simulink model "monocopter_sim"  (R2026a)
settings: Solver=ode4  StopTime=10  FixedStep=Ts
undefined symbols (not defined in the file): alt_ref_const, b_aero, b_pitch, b_roll, c_q, F_to_throttle, g, Ixx, Iyy, Izz, joy_pitch_const, joy_roll_const, kappa_y, Kd_alt, Kd_pitch, Kd_roll, Kd_yaw, Ki_alt, Ki_pitch, Ki_roll, Ki_yaw, Kp_alt, Kp_pitch, Kp_roll, Kp_yaw, Ks_hover, kT, Ky_hover, m, mode_const, omega_hover, omega_max, pid_alt_force_max, pid_alt_int_max, pid_pitch_int_max, pid_pitch_torque_max, pid_roll_int_max, pid_roll_torque_max, pid_yaw_int_max, pid_yaw_torque_max, servo_max, servo_min, throttle_const, Ts, yaw_ff, yaw_ref_const
libraries: slpidlib x4, simulink x4
settings Model: Creator=macbookpro
settings DataIOCC: SaveState=on

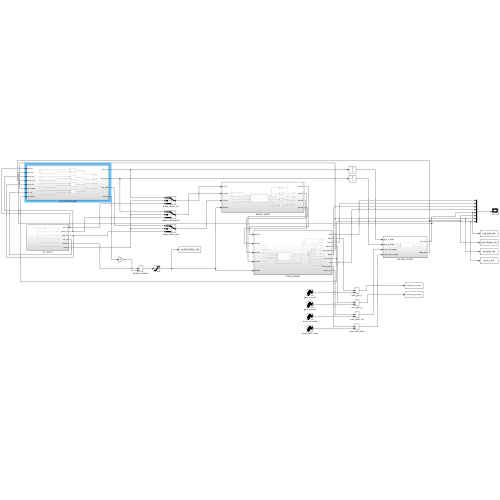
[thumbnail: Simulink's stored preview of the top-level diagram]
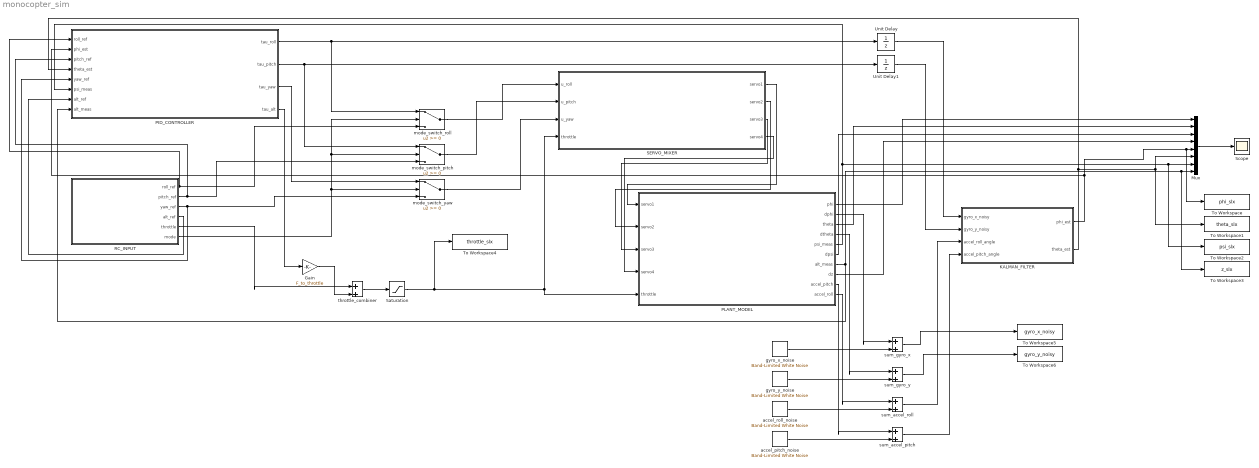
== system monocopter_sim ==
  Gain : Gain  Gain=F_to_throttle
  KALMAN_FILTER : Subsystem
  Mux : Mux  Inputs=8
  PID_CONTROLLER : Subsystem
  PLANT_MODEL : Subsystem
  RC_INPUT : Subsystem
  SERVO_MIXER : Subsystem
  Saturation : Saturate  UpperLimit=1  LowerLimit=0.05
  Scope : Scope
      settings: ActiveDisplayYMinimum=-8.14946670637509E+7  ActiveDisplayYMaximum=9.2907040776445866E+7
  To Workspace : ToWorkspace  VariableName=phi_slx  SaveFormat=Timeseries  SampleTime=-1
  To Workspace1 : ToWorkspace  VariableName=theta_slx  SaveFormat=Timeseries  SampleTime=-1
  To Workspace2 : ToWorkspace  VariableName=psi_slx  SaveFormat=Timeseries  SampleTime=-1
  To Workspace3 : ToWorkspace  VariableName=z_slx  SaveFormat=Timeseries  SampleTime=-1
  To Workspace4 : ToWorkspace  VariableName=throttle_slx  SaveFormat=Timeseries  SampleTime=-1
  To Workspace5 : ToWorkspace  VariableName=gyro_x_noisy  SaveFormat=Timeseries  SampleTime=-1
  To Workspace6 : ToWorkspace  VariableName=gyro_y_noisy  SaveFormat=Timeseries  SampleTime=-1
  Unit Delay : UnitDelay  SampleTime=Ts
  Unit Delay1 : UnitDelay  SampleTime=Ts
  "accel_pitch_noise " : simulink/Sources/Band-Limited White Noise  Cov=accel_noise_sim  Ts=Ts  seed=noise_seed_ap
  accel_roll_noise : simulink/Sources/Band-Limited White Noise  Cov=accel_noise_sim  Ts=Ts  seed=noise_seed_ar
  gyro_x_noise : simulink/Sources/Band-Limited White Noise  Cov=gyro_noise_sim  Ts=Ts  seed=noise_seed_gx
  gyro_y_noise : simulink/Sources/Band-Limited White Noise  Cov=gyro_noise_sim  Ts=Ts  seed=noise_seed_gy
  mode_switch_pitch : Switch  SaturateOnIntegerOverflow=off  InputSameDT=off
  mode_switch_roll : Switch  SaturateOnIntegerOverflow=off  InputSameDT=off
  mode_switch_yaw : Switch  SaturateOnIntegerOverflow=off  InputSameDT=off
  sum_accel_pitch : Sum  Inputs=|++
  sum_accel_roll : Sum  Inputs=|++
  sum_gyro_x : Sum  Inputs=|++
  sum_gyro_y : Sum  Inputs=|++
  throttle_combiner : Sum  Inputs=|++
  wires:
  PLANT_MODEL/2(dphi) -> sum_gyro_x/1
  gyro_x_noise/1 -> sum_gyro_x/2
  PLANT_MODEL/4(dtheta) -> sum_gyro_y/1
  gyro_y_noise/1 -> sum_gyro_y/2
  PLANT_MODEL/10(accel_roll) -> sum_accel_roll/1
  accel_roll_noise/1 -> sum_accel_roll/2
  PLANT_MODEL/9(accel_pitch) -> sum_accel_pitch/1
  "accel_pitch_noise "/1 -> sum_accel_pitch/2
  sum_accel_roll/1 -> KALMAN_FILTER/3(accel_roll_angle)
  sum_accel_pitch/1 -> KALMAN_FILTER/4(accel_pitch_angle)
  PID_CONTROLLER/1(tau_roll) -> Unit Delay/1, mode_switch_roll/1
  RC_INPUT/6(mode) -> mode_switch_yaw/2, mode_switch_roll/2, mode_switch_pitch/2
  RC_INPUT/1(roll_ref) -> PID_CONTROLLER/1(roll_ref), mode_switch_roll/3
  mode_switch_roll/1 -> SERVO_MIXER/1(u_roll)
  mode_switch_pitch/1 -> SERVO_MIXER/2(u_pitch)
  mode_switch_yaw/1 -> SERVO_MIXER/3(u_yaw)
  PID_CONTROLLER/2(tau_pitch) -> Unit Delay1/1, mode_switch_pitch/1
  PID_CONTROLLER/3(tau_yaw) -> mode_switch_yaw/1
  RC_INPUT/2(pitch_ref) -> PID_CONTROLLER/3(pitch_ref), mode_switch_pitch/3
  RC_INPUT/3(yaw_ref) -> PID_CONTROLLER/5(yaw_ref), mode_switch_yaw/3
  RC_INPUT/5(throttle) -> throttle_combiner/1
  RC_INPUT/4(alt_ref) -> PID_CONTROLLER/7(alt_ref)
  KALMAN_FILTER/1(phi_est) -> PID_CONTROLLER/2(phi_est), To Workspace/1, Mux/5
  KALMAN_FILTER/2(theta_est) -> Mux/6, To Workspace1/1, PID_CONTROLLER/4(theta_est)
  SERVO_MIXER/1(servo1) -> PLANT_MODEL/1(servo1)
  SERVO_MIXER/2(servo2) -> PLANT_MODEL/2(servo2)
  SERVO_MIXER/3(servo3) -> PLANT_MODEL/3(servo3)
  SERVO_MIXER/4(servo4) -> PLANT_MODEL/4(servo4)
  PLANT_MODEL/5(psi_meas) -> Mux/7, To Workspace2/1, PID_CONTROLLER/6(psi_meas)
  PLANT_MODEL/7(alt_meas) -> Mux/8, To Workspace3/1, PID_CONTROLLER/8(alt_meas)
  PLANT_MODEL/3(theta) -> Mux/2
  PLANT_MODEL/6(dpsi) -> Mux/3
  PLANT_MODEL/8(dz) -> Mux/4
  Mux/1 -> Scope/1
  PLANT_MODEL/1(phi) -> Mux/1
  throttle_combiner/1 -> Saturation/1
  Saturation/1 -> PLANT_MODEL/5(throttle), SERVO_MIXER/4(throttle), To Workspace4/1
  sum_gyro_y/1 -> To Workspace6/1
  PID_CONTROLLER/4(tau_alt) -> Gain/1
  Gain/1 -> throttle_combiner/2
  Unit Delay1/1 -> KALMAN_FILTER/2(gyro_y_noisy)
  sum_gyro_x/1 -> To Workspace5/1
  Unit Delay/1 -> KALMAN_FILTER/1(gyro_x_noisy)

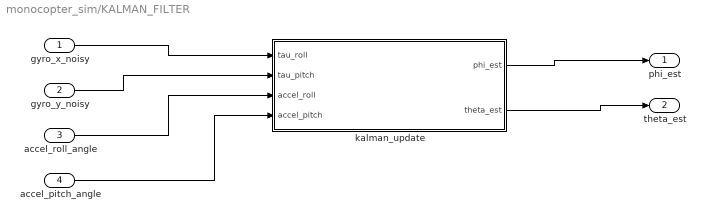
== system monocopter_sim/KALMAN_FILTER ==
  gyro_x_noisy : Inport
  gyro_y_noisy : Inport  Port=2
  accel_roll_angle : Inport  Port=3
  accel_pitch_angle : Inport  Port=4
  kalman_update : MATLAB Function  TreatAsAtomicUnit=on  SystemSampleTime=Ts
  phi_est : Outport
  theta_est : Outport  Port=2
  wires:
  gyro_x_noisy/1 -> kalman_update/1(tau_roll)
  gyro_y_noisy/1 -> kalman_update/2(tau_pitch)
  accel_roll_angle/1 -> kalman_update/3(accel_roll)
  accel_pitch_angle/1 -> kalman_update/4(accel_pitch)
  kalman_update/1(phi_est) -> phi_est/1
  kalman_update/2(theta_est) -> theta_est/1

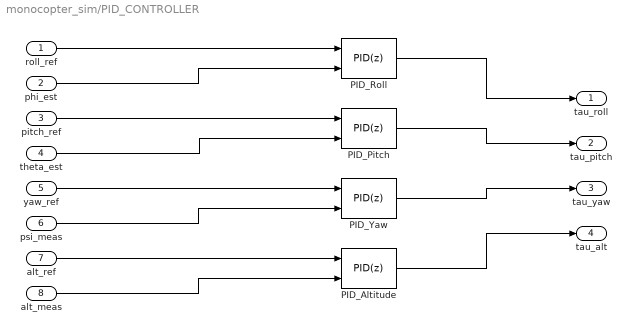
== system monocopter_sim/PID_CONTROLLER ==
  roll_ref : Inport
  phi_est : Inport  Port=2
  pitch_ref : Inport  Port=3
  theta_est : Inport  Port=4
  yaw_ref : Inport  Port=5
  psi_meas : Inport  Port=6
  alt_ref : Inport  Port=7
  alt_meas : Inport  Port=8
  PID_Altitude : slpidlib/PID Controller (2DOF)  Controller=PID  Form=Parallel  TimeDomain=Discrete-time  UseExternalTs=off  SampleTime=Ts  IntegratorMethod=Forward Euler  FilterMethod=Forward Euler  ControllerParametersSource=internal  P=Kp_alt  I=Ki_alt  UseKiTs=off  D=Kd_alt  UseExternalDerivativeSource=off  N=100  UseFilter=on  b=0  c=0  TunerSelectOption=Transfer Function Based (PID Tuner App)  InitialConditionSource=internal  InitialConditionForIntegrator=0  InitialConditionForFilter=0  DifferentiatorICPrevScaledInput=0  ExternalReset=none  TrackingMode=off  Kt=1  LimitOutput=on  SatLimitsSource=internal  UpperSaturationLimit=pid_alt_force_max  LowerSaturationLimit=-pid_alt_force_max  LinearizeAsGain=on  AntiWindupMode=clamping  Kb=1  LimitIntegrator=on  UpperIntegratorSaturationLimit=pid_alt_int_max  LowerIntegratorSaturationLimit=-pid_alt_int_max  POutMin=[]  POutMax=[]  IOutMin=[]  IOutMax=[]  DOutMin=[]  DOutMax=[]  NOutMin=[]  NOutMax=[]  bOutMin=[]  bOutMax=[]  cOutMin=[]  cOutMax=[]  SumOutMin=[]  SumOutMax=[]  SaturationOutMin=[]  SaturationOutMax=[]  PParamMin=[]  PParamMax=[]  IParamMin=[]  IParamMax=[]  DParamMin=[]  DParamMax=[]  NParamMin=[]  NParamMax=[]  bParamMin=[]  bParamMax=[]  cParamMin=[]  cParamMax=[]  KbParamMin=[]  KbParamMax=[]  KtParamMin=[]  KtParamMax=[]  KbOutMin=[]  KbOutMax=[]  KtOutMin=[]  KtOutMax=[]  IntegratorOutMin=[]  IntegratorOutMax=[]  FilterOutMin=[]  FilterOutMax=[]  SumI1OutMin=[]  SumI1OutMax=[]  SumI2OutMin=[]  SumI2OutMax=[]  SumI3OutMin=[]  SumI3OutMax=[]  SumI4OutMin=[]  SumI4OutMax=[]  SumDOutMin=[]  SumDOutMax=[]  Sum1OutMin=[]  Sum1OutMax=[]  Sum2OutMin=[]  Sum2OutMax=[]  Sum3OutMin=[]  Sum3OutMax=[]  DifferentiatorOutMin=[]  DifferentiatorOutMax=[]  FilterDiffOutCoefMin=[]  FilterDiffOutCoefMax=[]  ReciprocalOutMin=[]  ReciprocalOutMax=[]  SumDenOutMin=[]  SumDenOutMax=[]  SumNumOutMin=[]  SumNumOutMax=[]  DivideOutMin=[]  DivideOutMax=[]  UdiffTsProdOutMin=[]  UdiffTsProdOutMax=[]  NTsProdOutMin=[]  NTsProdOutMax=[]  UintegralTsProdOutMin=[]  UintegralTsProdOutMax=[]  UngainTsProdOutMin=[]  UngainTsProdOutMax=[]  ClampingZeroOutDataTypeStr=Inherit: Inherit via back propagation  ClampingZeroOutMin=[]  ClampingZeroOutMax=[]  FilterDenConstantOutDataTypeStr=Inherit: Inherit via back propagation  FilterDenConstantOutMin=[]  FilterDenConstantOutMax=[]  PCopyOutDataTypeStr=Inherit: Inherit via back propagation  PCopyOutMin=[]  PCopyOutMax=[]  NCopyOutDataTypeStr=Inherit: Inherit via back propagation  NCopyOutMin=[]  NCopyOutMax=[]  IntegratorContinuousStateAttributes=''  IntegratorStateMustResolveToSignalObject=off  IntegratorRTWStateStorageClass=Auto  FilterContinuousStateAttributes=''  FilterStateMustResolveToSignalObject=off  FilterRTWStateStorageClass=Auto  ParallelPVariant=InternalParameters  IdealPVariant=Disabled  IVariant=InternalParameters  DVariant=InternalParameters  bVariant=InternalParameters  cVariant=InternalParameters  IntegratorVariant=Discrete  SatVariant=Enabled  AWVariant=DiscClampingParallel  PCopyVariant=Disabled  TRVariant=Disabled  FdbkBlocksVariant=Forward  IdealPFdbkVariant=Disabled  SatFdbkVariant=Disabled  DerivativeFilterVariant=ForwardEulerFilter  NVariant=InternalParameters  NCopyVariant=Disabled  FilterICVariant=InternalICsFilter  IntegratorICVariant=InternalICs  ExternalResetVariant=Disabled  TRSumVariant=Passthrough  SumFdbkVariant=Disabled  SumVariant=Sum_PID  TsampFilterVariant=InternalTs  TsampNgainVariant=Passthrough  TsampIntegralVariant=Disabled_SignalSpec  ExternalSaturationOutDataTypeStr=Inherit: Same as second input  DerivativeSourceVariant=ErrorSignal  PreIntVariant=InternalPreInt
  PID_Pitch : slpidlib/PID Controller (2DOF)  Controller=PID  Form=Parallel  TimeDomain=Discrete-time  UseExternalTs=off  SampleTime=Ts  IntegratorMethod=Forward Euler  FilterMethod=Forward Euler  ControllerParametersSource=internal  P=Kp_pitch  I=Ki_pitch  UseKiTs=off  D=Kd_pitch  UseExternalDerivativeSource=off  N=100  UseFilter=on  b=0  c=0  TunerSelectOption=Transfer Function Based (PID Tuner App)  InitialConditionSource=internal  InitialConditionForIntegrator=0  InitialConditionForFilter=0  DifferentiatorICPrevScaledInput=0  ExternalReset=none  TrackingMode=off  Kt=1  LimitOutput=on  SatLimitsSource=internal  UpperSaturationLimit=pid_pitch_torque_max  LowerSaturationLimit=-pid_pitch_torque_max  LinearizeAsGain=on  AntiWindupMode=clamping  Kb=1  LimitIntegrator=on  UpperIntegratorSaturationLimit=pid_pitch_int_max  LowerIntegratorSaturationLimit=-pid_pitch_int_max  POutMin=[]  POutMax=[]  IOutMin=[]  IOutMax=[]  DOutMin=[]  DOutMax=[]  NOutMin=[]  NOutMax=[]  bOutMin=[]  bOutMax=[]  cOutMin=[]  cOutMax=[]  SumOutMin=[]  SumOutMax=[]  SaturationOutMin=[]  SaturationOutMax=[]  PParamMin=[]  PParamMax=[]  IParamMin=[]  IParamMax=[]  DParamMin=[]  DParamMax=[]  NParamMin=[]  NParamMax=[]  bParamMin=[]  bParamMax=[]  cParamMin=[]  cParamMax=[]  KbParamMin=[]  KbParamMax=[]  KtParamMin=[]  KtParamMax=[]  KbOutMin=[]  KbOutMax=[]  KtOutMin=[]  KtOutMax=[]  IntegratorOutMin=[]  IntegratorOutMax=[]  FilterOutMin=[]  FilterOutMax=[]  SumI1OutMin=[]  SumI1OutMax=[]  SumI2OutMin=[]  SumI2OutMax=[]  SumI3OutMin=[]  SumI3OutMax=[]  SumI4OutMin=[]  SumI4OutMax=[]  SumDOutMin=[]  SumDOutMax=[]  Sum1OutMin=[]  Sum1OutMax=[]  Sum2OutMin=[]  Sum2OutMax=[]  Sum3OutMin=[]  Sum3OutMax=[]  DifferentiatorOutMin=[]  DifferentiatorOutMax=[]  FilterDiffOutCoefMin=[]  FilterDiffOutCoefMax=[]  ReciprocalOutMin=[]  ReciprocalOutMax=[]  SumDenOutMin=[]  SumDenOutMax=[]  SumNumOutMin=[]  SumNumOutMax=[]  DivideOutMin=[]  DivideOutMax=[]  UdiffTsProdOutMin=[]  UdiffTsProdOutMax=[]  NTsProdOutMin=[]  NTsProdOutMax=[]  UintegralTsProdOutMin=[]  UintegralTsProdOutMax=[]  UngainTsProdOutMin=[]  UngainTsProdOutMax=[]  ClampingZeroOutDataTypeStr=Inherit: Inherit via back propagation  ClampingZeroOutMin=[]  ClampingZeroOutMax=[]  FilterDenConstantOutDataTypeStr=Inherit: Inherit via back propagation  FilterDenConstantOutMin=[]  FilterDenConstantOutMax=[]  PCopyOutDataTypeStr=Inherit: Inherit via back propagation  PCopyOutMin=[]  PCopyOutMax=[]  NCopyOutDataTypeStr=Inherit: Inherit via back propagation  NCopyOutMin=[]  NCopyOutMax=[]  IntegratorContinuousStateAttributes=''  IntegratorStateMustResolveToSignalObject=off  IntegratorRTWStateStorageClass=Auto  FilterContinuousStateAttributes=''  FilterStateMustResolveToSignalObject=off  FilterRTWStateStorageClass=Auto  ParallelPVariant=InternalParameters  IdealPVariant=Disabled  IVariant=InternalParameters  DVariant=InternalParameters  bVariant=InternalParameters  cVariant=InternalParameters  IntegratorVariant=Discrete  SatVariant=Enabled  AWVariant=DiscClampingParallel  PCopyVariant=Disabled  TRVariant=Disabled  FdbkBlocksVariant=Forward  IdealPFdbkVariant=Disabled  SatFdbkVariant=Disabled  DerivativeFilterVariant=ForwardEulerFilter  NVariant=InternalParameters  NCopyVariant=Disabled  FilterICVariant=InternalICsFilter  IntegratorICVariant=InternalICs  ExternalResetVariant=Disabled  TRSumVariant=Passthrough  SumFdbkVariant=Disabled  SumVariant=Sum_PID  TsampFilterVariant=InternalTs  TsampNgainVariant=Passthrough  TsampIntegralVariant=Disabled_SignalSpec  ExternalSaturationOutDataTypeStr=Inherit: Same as second input  DerivativeSourceVariant=ErrorSignal  PreIntVariant=InternalPreInt
  PID_Roll : slpidlib/PID Controller (2DOF)  Controller=PID  Form=Parallel  TimeDomain=Discrete-time  UseExternalTs=off  SampleTime=Ts  IntegratorMethod=Forward Euler  FilterMethod=Forward Euler  ControllerParametersSource=internal  P=Kp_roll  I=Ki_roll  UseKiTs=off  D=Kd_roll  UseExternalDerivativeSource=off  N=100  UseFilter=on  b=0  c=0  TunerSelectOption=Transfer Function Based (PID Tuner App)  InitialConditionSource=internal  InitialConditionForIntegrator=0  InitialConditionForFilter=0  DifferentiatorICPrevScaledInput=0  ExternalReset=none  TrackingMode=off  Kt=1  LimitOutput=on  SatLimitsSource=internal  UpperSaturationLimit=pid_roll_torque_max  LowerSaturationLimit=-pid_roll_torque_max  LinearizeAsGain=on  AntiWindupMode=clamping  Kb=1  LimitIntegrator=on  UpperIntegratorSaturationLimit=pid_roll_int_max  LowerIntegratorSaturationLimit=-pid_roll_int_max  POutMin=[]  POutMax=[]  IOutMin=[]  IOutMax=[]  DOutMin=[]  DOutMax=[]  NOutMin=[]  NOutMax=[]  bOutMin=[]  bOutMax=[]  cOutMin=[]  cOutMax=[]  SumOutMin=[]  SumOutMax=[]  SaturationOutMin=[]  SaturationOutMax=[]  PParamMin=[]  PParamMax=[]  IParamMin=[]  IParamMax=[]  DParamMin=[]  DParamMax=[]  NParamMin=[]  NParamMax=[]  bParamMin=[]  bParamMax=[]  cParamMin=[]  cParamMax=[]  KbParamMin=[]  KbParamMax=[]  KtParamMin=[]  KtParamMax=[]  KbOutMin=[]  KbOutMax=[]  KtOutMin=[]  KtOutMax=[]  IntegratorOutMin=[]  IntegratorOutMax=[]  FilterOutMin=[]  FilterOutMax=[]  SumI1OutMin=[]  SumI1OutMax=[]  SumI2OutMin=[]  SumI2OutMax=[]  SumI3OutMin=[]  SumI3OutMax=[]  SumI4OutMin=[]  SumI4OutMax=[]  SumDOutMin=[]  SumDOutMax=[]  Sum1OutMin=[]  Sum1OutMax=[]  Sum2OutMin=[]  Sum2OutMax=[]  Sum3OutMin=[]  Sum3OutMax=[]  DifferentiatorOutMin=[]  DifferentiatorOutMax=[]  FilterDiffOutCoefMin=[]  FilterDiffOutCoefMax=[]  ReciprocalOutMin=[]  ReciprocalOutMax=[]  SumDenOutMin=[]  SumDenOutMax=[]  SumNumOutMin=[]  SumNumOutMax=[]  DivideOutMin=[]  DivideOutMax=[]  UdiffTsProdOutMin=[]  UdiffTsProdOutMax=[]  NTsProdOutMin=[]  NTsProdOutMax=[]  UintegralTsProdOutMin=[]  UintegralTsProdOutMax=[]  UngainTsProdOutMin=[]  UngainTsProdOutMax=[]  ClampingZeroOutDataTypeStr=Inherit: Inherit via back propagation  ClampingZeroOutMin=[]  ClampingZeroOutMax=[]  FilterDenConstantOutDataTypeStr=Inherit: Inherit via back propagation  FilterDenConstantOutMin=[]  FilterDenConstantOutMax=[]  PCopyOutDataTypeStr=Inherit: Inherit via back propagation  PCopyOutMin=[]  PCopyOutMax=[]  NCopyOutDataTypeStr=Inherit: Inherit via back propagation  NCopyOutMin=[]  NCopyOutMax=[]  IntegratorContinuousStateAttributes=''  IntegratorStateMustResolveToSignalObject=off  IntegratorRTWStateStorageClass=Auto  FilterContinuousStateAttributes=''  FilterStateMustResolveToSignalObject=off  FilterRTWStateStorageClass=Auto  ParallelPVariant=InternalParameters  IdealPVariant=Disabled  IVariant=InternalParameters  DVariant=InternalParameters  bVariant=InternalParameters  cVariant=InternalParameters  IntegratorVariant=Discrete  SatVariant=Enabled  AWVariant=DiscClampingParallel  PCopyVariant=Disabled  TRVariant=Disabled  FdbkBlocksVariant=Forward  IdealPFdbkVariant=Disabled  SatFdbkVariant=Disabled  DerivativeFilterVariant=ForwardEulerFilter  NVariant=InternalParameters  NCopyVariant=Disabled  FilterICVariant=InternalICsFilter  IntegratorICVariant=InternalICs  ExternalResetVariant=Disabled  TRSumVariant=Passthrough  SumFdbkVariant=Disabled  SumVariant=Sum_PID  TsampFilterVariant=InternalTs  TsampNgainVariant=Passthrough  TsampIntegralVariant=Disabled_SignalSpec  ExternalSaturationOutDataTypeStr=Inherit: Same as second input  DerivativeSourceVariant=ErrorSignal  PreIntVariant=InternalPreInt
  PID_Yaw : slpidlib/PID Controller (2DOF)  Controller=PID  Form=Parallel  TimeDomain=Discrete-time  UseExternalTs=off  SampleTime=Ts  IntegratorMethod=Forward Euler  FilterMethod=Forward Euler  ControllerParametersSource=internal  P=Kp_yaw  I=Ki_yaw  UseKiTs=off  D=Kd_yaw  UseExternalDerivativeSource=off  N=100  UseFilter=on  b=0  c=0  TunerSelectOption=Transfer Function Based (PID Tuner App)  InitialConditionSource=internal  InitialConditionForIntegrator=0  InitialConditionForFilter=0  DifferentiatorICPrevScaledInput=0  ExternalReset=none  TrackingMode=off  Kt=1  LimitOutput=on  SatLimitsSource=internal  UpperSaturationLimit=pid_yaw_torque_max  LowerSaturationLimit=-pid_yaw_torque_max  LinearizeAsGain=on  AntiWindupMode=clamping  Kb=1  LimitIntegrator=on  UpperIntegratorSaturationLimit=pid_yaw_int_max  LowerIntegratorSaturationLimit=-pid_yaw_int_max  POutMin=[]  POutMax=[]  IOutMin=[]  IOutMax=[]  DOutMin=[]  DOutMax=[]  NOutMin=[]  NOutMax=[]  bOutMin=[]  bOutMax=[]  cOutMin=[]  cOutMax=[]  SumOutMin=[]  SumOutMax=[]  SaturationOutMin=[]  SaturationOutMax=[]  PParamMin=[]  PParamMax=[]  IParamMin=[]  IParamMax=[]  DParamMin=[]  DParamMax=[]  NParamMin=[]  NParamMax=[]  bParamMin=[]  bParamMax=[]  cParamMin=[]  cParamMax=[]  KbParamMin=[]  KbParamMax=[]  KtParamMin=[]  KtParamMax=[]  KbOutMin=[]  KbOutMax=[]  KtOutMin=[]  KtOutMax=[]  IntegratorOutMin=[]  IntegratorOutMax=[]  FilterOutMin=[]  FilterOutMax=[]  SumI1OutMin=[]  SumI1OutMax=[]  SumI2OutMin=[]  SumI2OutMax=[]  SumI3OutMin=[]  SumI3OutMax=[]  SumI4OutMin=[]  SumI4OutMax=[]  SumDOutMin=[]  SumDOutMax=[]  Sum1OutMin=[]  Sum1OutMax=[]  Sum2OutMin=[]  Sum2OutMax=[]  Sum3OutMin=[]  Sum3OutMax=[]  DifferentiatorOutMin=[]  DifferentiatorOutMax=[]  FilterDiffOutCoefMin=[]  FilterDiffOutCoefMax=[]  ReciprocalOutMin=[]  ReciprocalOutMax=[]  SumDenOutMin=[]  SumDenOutMax=[]  SumNumOutMin=[]  SumNumOutMax=[]  DivideOutMin=[]  DivideOutMax=[]  UdiffTsProdOutMin=[]  UdiffTsProdOutMax=[]  NTsProdOutMin=[]  NTsProdOutMax=[]  UintegralTsProdOutMin=[]  UintegralTsProdOutMax=[]  UngainTsProdOutMin=[]  UngainTsProdOutMax=[]  ClampingZeroOutDataTypeStr=Inherit: Inherit via back propagation  ClampingZeroOutMin=[]  ClampingZeroOutMax=[]  FilterDenConstantOutDataTypeStr=Inherit: Inherit via back propagation  FilterDenConstantOutMin=[]  FilterDenConstantOutMax=[]  PCopyOutDataTypeStr=Inherit: Inherit via back propagation  PCopyOutMin=[]  PCopyOutMax=[]  NCopyOutDataTypeStr=Inherit: Inherit via back propagation  NCopyOutMin=[]  NCopyOutMax=[]  IntegratorContinuousStateAttributes=''  IntegratorStateMustResolveToSignalObject=off  IntegratorRTWStateStorageClass=Auto  FilterContinuousStateAttributes=''  FilterStateMustResolveToSignalObject=off  FilterRTWStateStorageClass=Auto  ParallelPVariant=InternalParameters  IdealPVariant=Disabled  IVariant=InternalParameters  DVariant=InternalParameters  bVariant=InternalParameters  cVariant=InternalParameters  IntegratorVariant=Discrete  SatVariant=Enabled  AWVariant=DiscClampingParallel  PCopyVariant=Disabled  TRVariant=Disabled  FdbkBlocksVariant=Forward  IdealPFdbkVariant=Disabled  SatFdbkVariant=Disabled  DerivativeFilterVariant=ForwardEulerFilter  NVariant=InternalParameters  NCopyVariant=Disabled  FilterICVariant=InternalICsFilter  IntegratorICVariant=InternalICs  ExternalResetVariant=Disabled  TRSumVariant=Passthrough  SumFdbkVariant=Disabled  SumVariant=Sum_PID  TsampFilterVariant=InternalTs  TsampNgainVariant=Passthrough  TsampIntegralVariant=Disabled_SignalSpec  ExternalSaturationOutDataTypeStr=Inherit: Same as second input  DerivativeSourceVariant=ErrorSignal  PreIntVariant=InternalPreInt
  tau_roll : Outport
  tau_pitch : Outport  Port=2
  tau_yaw : Outport  Port=3
  tau_alt : Outport  Port=4
  wires:
  roll_ref/1 -> PID_Roll/1
  phi_est/1 -> PID_Roll/2
  PID_Roll/1 -> tau_roll/1
  pitch_ref/1 -> PID_Pitch/1
  theta_est/1 -> PID_Pitch/2
  PID_Pitch/1 -> tau_pitch/1
  yaw_ref/1 -> PID_Yaw/1
  psi_meas/1 -> PID_Yaw/2
  PID_Yaw/1 -> tau_yaw/1
  alt_ref/1 -> PID_Altitude/1
  alt_meas/1 -> PID_Altitude/2
  PID_Altitude/1 -> tau_alt/1

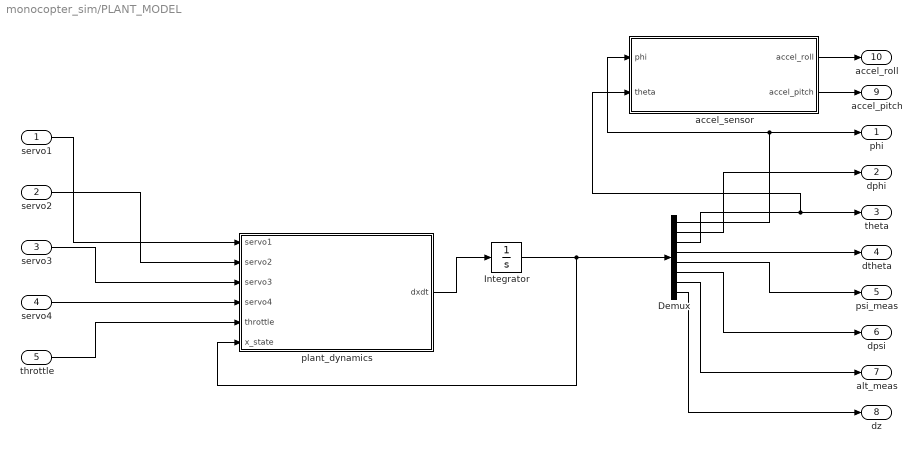
== system monocopter_sim/PLANT_MODEL ==
  servo1 : Inport  OutDataTypeStr=double
  servo2 : Inport  Port=2  OutDataTypeStr=double
  servo3 : Inport  Port=3  OutDataTypeStr=double
  servo4 : Inport  Port=4  OutDataTypeStr=double
  throttle : Inport  Port=5  OutDataTypeStr=double
  Demux : Demux  Outputs=8
  Integrator : Integrator  InitialCondition=zeros(8,1)
  accel_sensor : MATLAB Function  TreatAsAtomicUnit=on
  plant_dynamics : MATLAB Function  TreatAsAtomicUnit=on
  phi : Outport
  dphi : Outport  Port=2
  theta : Outport  Port=3
  dtheta : Outport  Port=4
  psi_meas : Outport  Port=5
  dpsi : Outport  Port=6
  alt_meas : Outport  Port=7
  dz : Outport  Port=8
  accel_pitch : Outport  Port=9
  accel_roll : Outport  Port=10
  wires:
  Demux/1 -> phi/1, accel_sensor/1(phi)
  Demux/2 -> dphi/1
  Demux/3 -> theta/1, accel_sensor/2(theta)
  Demux/4 -> dtheta/1
  Demux/5 -> psi_meas/1
  Demux/6 -> dpsi/1
  Demux/7 -> alt_meas/1
  Demux/8 -> dz/1
  servo1/1 -> plant_dynamics/1(servo1)
  servo2/1 -> plant_dynamics/2(servo2)
  servo3/1 -> plant_dynamics/3(servo3)
  servo4/1 -> plant_dynamics/4(servo4)
  throttle/1 -> plant_dynamics/5(throttle)
  plant_dynamics/1(dxdt) -> Integrator/1
  Integrator/1 -> Demux/1, plant_dynamics/6(x_state)
  accel_sensor/1(accel_roll) -> accel_roll/1
  accel_sensor/2(accel_pitch) -> accel_pitch/1

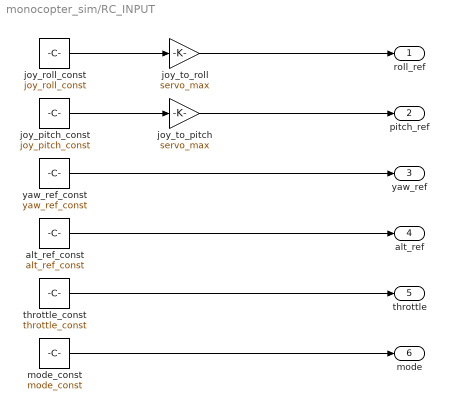
== system monocopter_sim/RC_INPUT ==
  alt_ref_const : Constant  Value=alt_ref_const  OutDataTypeStr=double
  joy_pitch_const : Constant  Value=joy_pitch_const  OutMin=[-1.0]  OutMax=[1.0]  OutDataTypeStr=double
  joy_roll_const : Constant  Value=joy_roll_const  OutMin=[-1.0]  OutMax=[1.0]  OutDataTypeStr=double
  joy_to_pitch : Gain  Gain=servo_max
  joy_to_roll : Gain  Gain=servo_max
  mode_const : Constant  Value=mode_const  OutMin=[0.0]  OutMax=[2.0]  OutDataTypeStr=double
  throttle_const : Constant  Value=throttle_const  OutMin=[0.0]  OutMax=[1.0]  OutDataTypeStr=double
  yaw_ref_const : Constant  Value=yaw_ref_const  OutDataTypeStr=double
  roll_ref : Outport
  pitch_ref : Outport  Port=2
  yaw_ref : Outport  Port=3
  alt_ref : Outport  Port=4
  throttle : Outport  Port=5
  mode : Outport  Port=6
  wires:
  joy_roll_const/1 -> joy_to_roll/1
  joy_to_roll/1 -> roll_ref/1
  joy_to_pitch/1 -> pitch_ref/1
  joy_pitch_const/1 -> joy_to_pitch/1
  throttle_const/1 -> throttle/1
  yaw_ref_const/1 -> yaw_ref/1
  alt_ref_const/1 -> alt_ref/1
  mode_const/1 -> mode/1

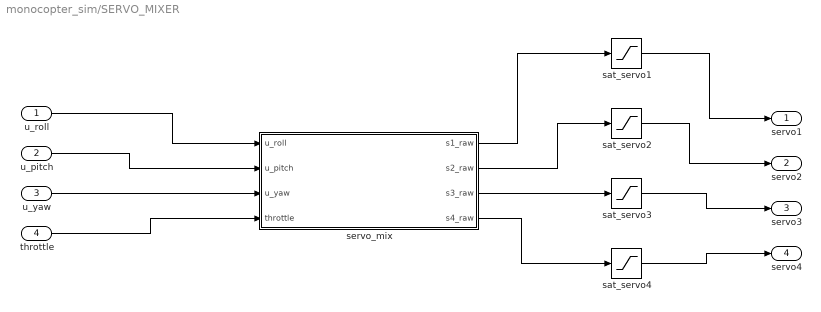
== system monocopter_sim/SERVO_MIXER ==
  u_roll : Inport
  u_pitch : Inport  Port=2
  u_yaw : Inport  Port=3
  throttle : Inport  Port=4
  sat_servo{1..4} (4 alike) : Saturate  UpperLimit=servo_max  LowerLimit=servo_min
  servo_mix : MATLAB Function  TreatAsAtomicUnit=on  SystemSampleTime=Ts
  servo1 : Outport
  servo2 : Outport  Port=2
  servo3 : Outport  Port=3
  servo4 : Outport  Port=4
  wires:
  u_roll/1 -> servo_mix/1(u_roll)
  u_pitch/1 -> servo_mix/2(u_pitch)
  u_yaw/1 -> servo_mix/3(u_yaw)
  servo_mix/1(s1_raw) -> sat_servo1/1
  servo_mix/2(s2_raw) -> sat_servo2/1
  servo_mix/3(s3_raw) -> sat_servo3/1
  servo_mix/4(s4_raw) -> sat_servo4/1
  sat_servo1/1 -> servo1/1
  sat_servo2/1 -> servo2/1
  sat_servo3/1 -> servo3/1
  sat_servo4/1 -> servo4/1
  throttle/1 -> servo_mix/4(throttle)

== matlab function monocopter_sim/PLANT_MODEL/accel_sensor ==
  data: phi input; accel_roll output; theta input; accel_pitch output
% accel_sensor — MATLAB Function Block

function [accel_roll, accel_pitch] = accel_sensor(phi, theta)

% Mensimulasikan pembacaan sudut dari accelerometer

% Di dunia nyata: sudut dihitung dari atan2(ay, sqrt(ax²+az²))

% Di simulasi: kita tahu phi dan theta langsung dari state


% Tambahkan sedikit noise accelerometer (disimulasikan terpisah dengan Band-Lim Noise)

% Di sini kita kembalikan sudut 'ideal' dari state

% Noise akan ditambahkan oleh blok Sum + Band-Limited White Noise di luar

accel_roll  = phi;    % Sudut roll dari akselerasi gravitasi

accel_pitch = theta;  % Sudut pitch dari akselerasi gravitasi


% Catatan fisik:

% Dalam implementasi ESP32 nyata, ini dihitung dari:

%   accel_roll  = atan2(ay, az)

%   accel_pitch = atan2(-ax, sqrt(ay^2 + az^2))

== matlab function monocopter_sim/PLANT_MODEL/plant_dynamics ==
  data: servo1 input; dxdt output; servo2 input; servo3 input; servo4 input; throttle input; x_state input; m parameter; g parameter; Ixx parameter; Iyy parameter; Izz parameter; kT parameter; Ks_hover parameter; omega_max parameter; b_aero parameter; c_q parameter; kappa_y parameter; omega_hover parameter
function dxdt = plant_dynamics(servo1, servo2, servo3, servo4, throttle, x_state, m, g, Ixx, Iyy, Izz, kT, Ks_hover, omega_max, b_aero, c_q, kappa_y, omega_hover)
%% ============================================================
%% plant_dynamics — MATLAB Function block untuk PLANT_MODEL
%% Model torsi sirip LINEAR (Ks_hover) — KONSISTEN dengan:
%%   monochopter_params.m, simulasi_full_system.m, BAB II/III
%% DIPERBARUI (v3, REVISI BAB III): HANYA penamaan parameter
%%   Keff -> Ks_hover untuk konsistensi notasi dengan Bab II/III
%%   (Ks_hover === Keff, nilai dan LOGIKA TIDAK BERUBAH dari v2 --
%%   plant_dynamics.m sejak awal sudah benar menghitung torsi FISIK
%%   Ks_hover*w(omega)*(delta1-delta3), dst., karena servo1..4 di
%%   sini adalah SUDUT FISIK aktual sirip setelah konversi torsi-ke-
%%   defleksi yang kini dilakukan di servo_mix.m v3, bukan di sini).
%% ============================================================
%
% INPUT:
%   servo1..4  : defleksi sirip [rad]   (dari SERVO_MIXER, SUDAH
%                dikonversi dari torsi ke radian di servo_mix.m v3)
%   throttle   : 0..1                    (dari throttle_combiner)
%   x_state    : [phi;dphi;theta;dtheta;psi;dpsi;z;dz]  (umpan balik 1/s)
%   Ks_hover   : efektivitas torsi sirip roll/pitch [N.m/rad] (dahulu Keff)
%   c_q        : koefisien torsi reaksi propeller [m]
%   kappa_y    : faktor efektivitas mixing kolektif yaw [-]
%   omega_hover: kecepatan sudut motor saat hover [rad/s] (referensi w)
% OUTPUT:
%   dxdt       : turunan state (8x1)
%
% CATATAN: Parameter dideklarasikan sebagai PARAMETER ARGUMENT.
%   Di "Ports and Data Manager" (Edit Data), set m, g, Ixx, Iyy, Izz,
%   kT, Ks_hover, omega_max, b_aero, c_q, kappa_y, omega_hover sebagai
%   Scope=Parameter agar otomatis terbaca dari workspace (hasil
%   monochopter_params.m v3, yang menyediakan Ks_hover langsung
%   sekaligus alias Keff untuk kompatibilitas mundur bila diperlukan).

%#codegen

% --- Unpack state --- 
phi   = x_state(1);  dphi   = x_state(2);
theta = x_state(3);  dtheta = x_state(4);
psi   = x_state(5);  dpsi   = x_state(6);
z     = x_state(7);  dz     = x_state(8);

% --- Gaya angkat motor --- 
omega = throttle * omega_max;
FT    = kT * omega^2;

% --- Torsi reaksi propeller (Hukum III Newton) --- 
% Q berlawanan arah putar propeller (CW propeller -> badan cenderung
% CCW, temuan uji terbang). Proporsional terhadap thrust AKTUAL
% (bervariasi dengan throttle) -- berbeda dari yaw_ff di servo_mix.m
% yang konstan (dihitung pada titik hover), sehingga residu gangguan
% di luar throttle hover akan tampak dan ditangani aksi integral PID_yaw.
Q_reaction = c_q * FT;

% --- Efektivitas sirip terhadap prop wash: w(omega) --- 
% downwash lebih kencang di throttle tinggi -> sirip dgn sudut SAMA
% menghasilkan torsi JAUH lebih besar. w=1 tepat di throttle hover
% (kalibrasi Ks_hover dilakukan di titik ini).
w_omega = (omega/omega_hover)^2;

% --- Torsi sirip: MODEL LINEAR Ks_hover*w(omega)*kappa_y + torsi
%     reaksi + redaman. Kompensasi gain-scheduling (1/w_omega) DAN
%     konversi torsi-ke-defleksi (1/(2*Ks_hover) atau 1/(4*Ky_hover))
%     SUDAH dilakukan di servo_mix.m v3 SEBELUM sampai di sini --
%     jadi servo1..4 di sini adalah SUDUT FISIK aktual sirip, dan
%     w_omega di baris tau_* menghasilkan torsi FISIK yang benar-
%     benar dihasilkan sirip pada kondisi throttle aktual (bukan
%     mengulang kompensasi yang sama untuk kedua kalinya). --- 
tau_roll  = Ks_hover*w_omega*(servo1 - servo3) - b_aero*dphi;
tau_pitch = Ks_hover*w_omega*(servo2 - servo4) - b_aero*dtheta;
tau_yaw   = Ks_hover*w_omega*kappa_y*(servo1+servo2+servo3+servo4) - Q_reaction - b_aero*dpsi;

% --- Persamaan Euler (rotasi benda tegar) --- 
ddphi   = ((Iyy-Izz)*dtheta*dpsi + tau_roll ) / Ixx;
ddtheta = ((Izz-Ixx)*dphi  *dpsi + tau_pitch) / Iyy;
ddpsi   = ((Ixx-Iyy)*dphi*dtheta + tau_yaw  ) / Izz;

% --- Translasi vertikal (Newton) --- 
ddz = -g + cos(phi)*cos(theta)*FT/m;

% --- Saturasi fisik (mencegah divergensi numerik) --- 
ddphi   = max(-150, min(150, ddphi));
ddtheta = max(-150, min(150, ddtheta));
ddpsi   = max(-80,  min(80,  ddpsi));
ddz     = max(-15,  min(15,  ddz));

% --- Susun turunan state --- 
dxdt = [dphi; ddphi; dtheta; ddtheta; dpsi; ddpsi; dz; ddz];

% Ground constraint (tidak menembus tanah)
if z <= 0 && dz < 0
    dxdt(7) = 0;
    dxdt(8) = max(0, dxdt(8));
end
end

== matlab function monocopter_sim/KALMAN_FILTER/kalman_update ==
  data: tau_roll input; phi_est output; tau_pitch input; accel_roll input; accel_pitch input; theta_est output; b_roll parameter; b_pitch parameter
% kalman_update — MATLAB Function Block

function [phi_est, theta_est] = kalman_update(tau_roll, tau_pitch, accel_roll, accel_pitch, b_roll, b_pitch)

% ============================================================

% KALMAN FILTER — Estimasi sudut Roll dan Pitch

% Menggunakan Discrete Kalman Filter

% DIPERBARUI (v3, REVISI BAB III Subbab 3.4-3.5): model proses kini

% memakai TORSI KENDALI (tau_roll, tau_pitch) siklus sebelumnya sebagai

% masukan u, BUKAN pembacaan giroskop langsung seperti v2. Perubahan

% ini menyatukan model proses DKF dengan model state-space fisik yang

% sama yang dipakai perancangan PID pole-placement (Bab II Subbab

% state-space, Bab III Subbab 3.4), sehingga tidak ada dua model

% berbeda untuk sistem yang sama.

%

% KONSEKUENSI: giroskop (gyro_x, gyro_y) TIDAK LAGI menjadi masukan

% fungsi ini -- sinyal giroskop tetap direkam ke workspace di kanvas

% top-level untuk keperluan pembanding (Bab IV), namun tidak masuk ke

% rekursi Kalman. Lihat Bab III Subbab arsitektur kendali untuk

% pembahasan keterbatasan metodologis pilihan desain ini.

% ============================================================

% PENJELASAN VARIABEL:

%   tau_roll    = torsi kendali roll siklus sebelumnya [N.m] (dari PID_CONTROLLER)

%   tau_pitch   = torsi kendali pitch siklus sebelumnya [N.m]

%   accel_roll  = sudut roll dari accelerometer [rad] (noisy, bisa drift)

%   accel_pitch = sudut pitch dari accelerometer [rad] (noisy, bisa drift)

%   b_roll      = 1/Ixx [rad/s^2 per N.m] (Parameter Argument, dari monochopter_params.m)

%   b_pitch     = 1/Iyy [rad/s^2 per N.m] (= b_roll karena Ixx=Iyy, tetap
%                 diberikan terpisah untuk keumuman/keterbacaan)

%   phi_est     = estimasi sudut roll [rad] (hasil filter, bersih)

%   theta_est   = estimasi sudut pitch [rad] (hasil filter, bersih)


% persistent: variabel yang bertahan nilainya antar pemanggilan fungsi

persistent x_roll P_roll x_pitch P_pitch initialized


% --- Inisialisasi saat pertama kali dipanggil --------------

if isempty(initialized)

    x_roll  = [0; 0];  % State roll awal: [sudut=0; rate=0]

    P_roll  = eye(2);  % Error covariance awal = identitas

    x_pitch = [0; 0];

    P_pitch = eye(2);

    initialized = true;

end


% --- Parameter Kalman (HARUS sama dengan params.m) --------

dt  = 0.005;                       % Sample time [s]

Q   = diag([0.001, 0.003]);       % Process noise: [angle_noise; rate_noise]

R   = 0.03;                        % Measurement noise (accelerometer)


% --- Matriks State-Space (BARU v3: berbasis TORSI, bukan kinematik) --

% State: [sudut; angular_rate]

% Model: sudut_baru = sudut_lama + dt*rate ; rate_baru = rate_lama + dt*b*tau

% (identik dengan Persamaan diskretisasi eksak Bab II/III, integrator

% ganda dgn gain fisik b=1/I -- BUKAN lagi model kinematik B=[0;dt]

% dengan u=giroskop seperti v2)

A = [1, dt; 0, 1];              % State transition matrix (TIDAK berubah dari v2)

C = [1, 0];                      % Observation matrix (hanya sudut yang diukur accel, TIDAK berubah)

B_roll  = [dt^2/2*b_roll;  dt*b_roll];   % BARU v3, menggantikan B=[0;dt] v2

B_pitch = [dt^2/2*b_pitch; dt*b_pitch];  % BARU v3


% ============================================================

% === ROLL KALMAN FILTER =====================================

% ============================================================


% --- STEP 1: PREDICT --------------------------------------

x_roll_pred = A * x_roll + B_roll * tau_roll;  % Prediksi state (BARU: masukan torsi)

P_roll_pred = A * P_roll * A' + Q;              % Prediksi error covariance


% --- STEP 2: UPDATE ---------------------------------------

S_r = C * P_roll_pred * C' + R;              % Innovation covariance

K_r = P_roll_pred * C' / S_r;               % Kalman Gain

innovation_r = accel_roll - C * x_roll_pred; % Residual (perbedaan pred vs ukur)

x_roll  = x_roll_pred + K_r * innovation_r;  % Update state

P_roll  = (eye(2) - K_r * C) * P_roll_pred; % Update error covariance


% --- Output roll -----------------------------------------

phi_est = x_roll(1);  % Ambil elemen pertama = estimasi sudut


% ============================================================

% === PITCH KALMAN FILTER ====================================

% ============================================================


% --- STEP 1: PREDICT --------------------------------------

x_pitch_pred = A * x_pitch + B_pitch * tau_pitch;  % BARU: masukan torsi

P_pitch_pred = A * P_pitch * A' + Q;

% --- STEP 2: UPDATE ---------------------------------------

S_p = C * P_pitch_pred * C' + R;

K_p = P_pitch_pred * C' / S_p;

innovation_p = accel_pitch - C * x_pitch_pred;

x_pitch  = x_pitch_pred + K_p * innovation_p;

P_pitch  = (eye(2) - K_p * C) * P_pitch_pred;


% --- Output pitch -----------------------------------------

theta_est = x_pitch(1);

end

== matlab function monocopter_sim/SERVO_MIXER/servo_mix ==
  data: u_roll input; s1_raw output; u_pitch input; u_yaw input; yaw_ff parameter; s2_raw output; s3_raw output; s4_raw output; throttle input; omega_max parameter; omega_hover parameter; Ks_hover parameter; Ky_hover parameter
% servo_mix — MATLAB Function Block

function [s1_raw, s2_raw, s3_raw, s4_raw] = servo_mix(u_roll, u_pitch, u_yaw, yaw_ff, throttle, omega_max, omega_hover, Ks_hover, Ky_hover)

  % ============================================================

  % SERVO MIXER — Monochopter 4-Servo

  % DIPERBARUI (v3, REVISI BAB III Subbab 3.7-3.8): u_roll/u_pitch/
  % u_yaw kini bersatuan TORSI MURNI (N.m), bukan lagi setara-sudut-
  % sirip seperti v2. Akibatnya, SETELAH kompensasi gain-scheduling
  % 1/w(omega), diperlukan LANGKAH TAMBAHAN yang v2 TIDAK punya:
  % konversi torsi-ke-defleksi dengan membagi Ks_hover (roll/pitch)
  % atau Ky_hover (yaw). Tanpa langkah ini, sirip akan menerima
  % perintah defleksi yang jauh lebih besar dari yang seharusnya
  % (karena Kp/Ki/Kd v3 baru jauh lebih besar nilainya, satuan N.m/rad
  % bukan rad/rad -- lihat monochopter_params.m v3).
  %
  % Urutan operasi (WAJIB dalam urutan ini):
  %   1) bagi w(omega)          -> kompensasi gain-scheduling (spt v2)
  %   2) bagi 2*Ks_hover / 4*Ky_hover -> konversi torsi ke radian (BARU v3)
  %   3) jumlahkan yaw_ff (kolektif, TIDAK ikut langkah 1 & 2 -- sudah
  %      dihitung dalam satuan radian sejak monochopter_params.m)
  %
  % Ks_hover, Ky_hover ditambahkan sebagai Parameter Argument baru
  % (Ports and Data Manager), dengan cara yang SAMA seperti Keff/
  % omega_hover sebelumnya (Ks_hover menggantikan peran Keff di sini;
  % Ky_hover = kappa_y*Ks_hover, sudah dihitung di monochopter_params.m).
  %
  % CATATAN PENTING (TIDAK BERUBAH dari v2): yaw_ff TIDAK ikut dibagi
  % w(omega) maupun Ks_hover/Ky_hover -- yaw_ff sudah final dalam
  % satuan RADIAN sejak dihitung di monochopter_params.m
  % (yaw_ff = Q_hover/(4*Ky_hover)), karena Q(omega) dan w(omega)
  % sama-sama berskala omega^2 sehingga rasionya otomatis konstan.

  % ============================================================

  % Layout fisik servo (dilihat dari atas):

  %

  %         DEPAN

  %          [S2]          ← Servo 2, posisi 0° (depan)

  %   [S1]   [M]   [S3]   ← Servo 1 kiri (270°), Motor tengah, Servo 3 kanan (90°)

  %          [S4]          ← Servo 4, posisi 180° (belakang)

  %         BELAKANG

  %

  % Logika mixing:

  %   ROLL  kanan (+): S1 defleksi -, S3 defleksi +  → wahana miring kanan

  %   PITCH maju  (+): S2 defleksi +, S4 defleksi -  → wahana miring depan

  %   YAW   searah (+): semua servo defleksi searah   → wahana berputar

  %   YAW_FF: bias kolektif KONSTAN (titik hover) menawar torsi reaksi

  %   propeller -- sirip TIDAK PERNAH netral saat hover (biaya permanen

  %   konfigurasi single-rotor, lihat BAB II/IV)


  % --- Langkah 1: Gain scheduling -- efektivitas sirip vs throttle ---
  omega   = throttle * omega_max;
  w_omega = (omega/omega_hover)^2;
  w_omega = max(w_omega, 0.05);   % guard pembagian oleh nilai sangat kecil
                                   % saat throttle rendah/motor idle

  u_roll_c  = u_roll  / w_omega;   % masih TORSI (N.m), belum jadi sudut
  u_pitch_c = u_pitch / w_omega;
  u_yaw_c   = u_yaw   / w_omega;

  % --- Langkah 2 (BARU v3): Konversi torsi-ke-defleksi ---
  % delta = torsi / (efektivitas sirip), menghasilkan RADIAN sirip.
  delta_roll  = u_roll_c  / (2*Ks_hover);
  delta_pitch = u_pitch_c / (2*Ks_hover);
  delta_yaw   = u_yaw_c   / (4*Ky_hover);

  % --- Langkah 3: Mixing matrix + feedforward kolektif ---

  % Format: s = M * [delta_roll; delta_pitch; delta_yaw] + yaw_ff
  % (yaw_ff sudah dalam satuan radian, TANPA kompensasi tambahan)

  s1_raw =  delta_roll  +  0           +  delta_yaw  +  yaw_ff;   % Servo 1 (kiri, 270°)

  s2_raw =  0           +  delta_pitch +  delta_yaw  +  yaw_ff;   % Servo 2 (depan, 0°)

  s3_raw = -delta_roll  +  0           +  delta_yaw  +  yaw_ff;   % Servo 3 (kanan, 90°)

  s4_raw =  0           + -delta_pitch +  delta_yaw  +  yaw_ff;   % Servo 4 (belakang, 180°)


  % CATATAN: Saturation (clamp ±servo_max) dilakukan di Saturation block

  % yang terpisah, bukan di sini. Ini memudahkan monitoring nilai sebelum saturasi.
end
